simulink model "double_PID_actual"  (R2024b)
settings: Solver=VariableStepAuto  StartTime=0  StopTime=3  FixedStep=0.0000001
undefined symbols (not defined in the file or in its folder): DiscIntNeverNeededParam
libraries: simulink x6
settings Model: Creator=kentl  LastModifiedBy=kentliukx

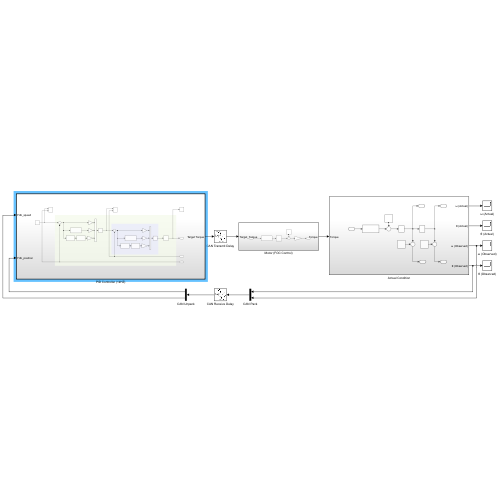
[thumbnail: Simulink's stored preview of the top-level diagram]
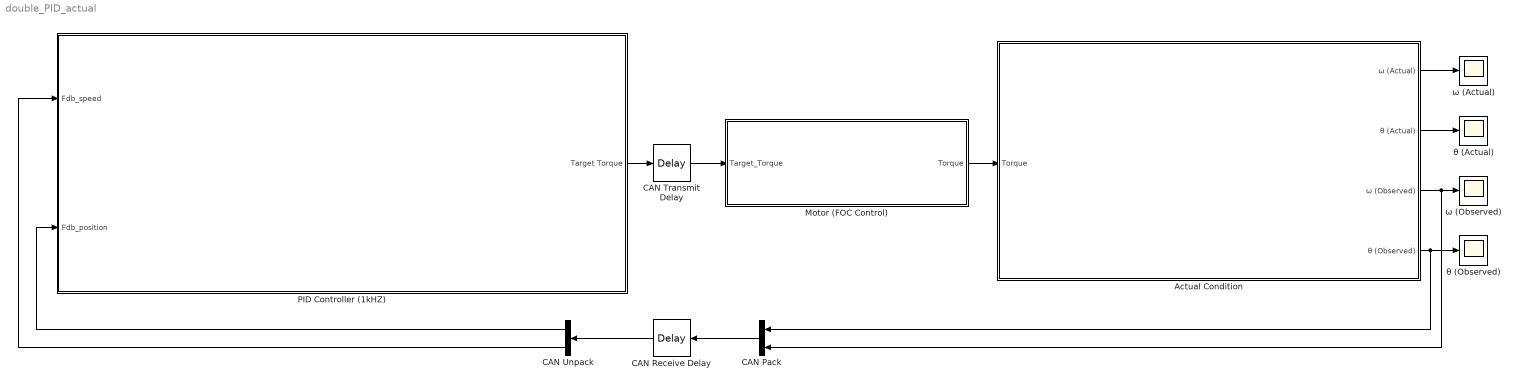
== system double_PID_actual ==
  "Actual Condition " : Subsystem
  CAN Pack : Mux  Inputs=2
  CAN Receive Delay : TransportDelay  DelayTime=0.001
  CAN Transmit Delay : TransportDelay  DelayTime=0.001
  CAN Unpack : Demux  Outputs=2
  "Motor (FOC Control) " : Subsystem
  "PID Controller (1kHZ) " : Subsystem  TreatAsAtomicUnit=on  PartitionName=PID  SystemSampleTime=0.001
  θ (Actual) : Scope
  θ (Observed) : Scope
  ω (Actual) : Scope
  ω (Observed) : Scope
  wires:
  CAN Pack/1 -> CAN Receive Delay/1
  CAN Receive Delay/1 -> CAN Unpack/1
  CAN Unpack/2 -> "PID Controller (1kHZ) "/1(Fdb_speed)
  CAN Unpack/1 -> "PID Controller (1kHZ) "/2(Fdb_position)
  "PID Controller (1kHZ) "/1(Target Torque) -> CAN Transmit Delay/1
  CAN Transmit Delay/1 -> "Motor (FOC Control) "/1(Target_Torque)
  "Actual Condition "/1(ω (Actual)) -> ω (Actual)/1
  "Actual Condition "/2(θ (Actual)) -> θ (Actual)/1
  "Actual Condition "/3(ω (Observed)) -> ω (Observed)/1, CAN Pack/2
  "Actual Condition "/4(θ (Observed)) -> θ (Observed)/1, CAN Pack/1
  "Motor (FOC Control) "/1(Torque) -> "Actual Condition "/1(Torque)

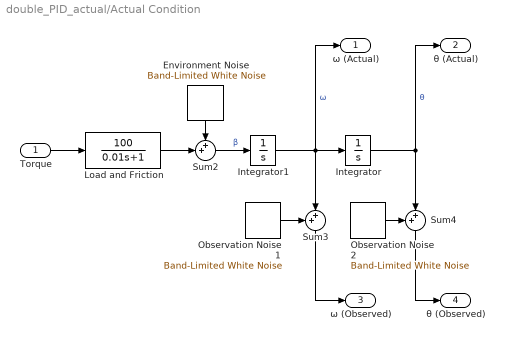
== system double_PID_actual/Actual Condition  ==
  Torque : Inport
  Environment Noise : simulink/Sources/Band-Limited White Noise  Cov=0.1  Ts=0.001  seed=[2331]
  Integrator : Integrator
  Integrator1 : Integrator
  Load and Friction : TransferFcn  Numerator=[100]  Denominator=[0.01 1]
  Observation Noise 1 : simulink/Sources/Band-Limited White Noise  Cov=0.0000001  Ts=0.001  seed=[23341]
  Observation Noise 2 : simulink/Sources/Band-Limited White Noise  Cov=0.0000001  Ts=0.001  seed=[23340]
  Sum2 : Sum  Inputs=++|
  Sum3 : Sum  Inputs=++|
  Sum4 : Sum  Inputs=++|
  ω (Actual) : Outport
  θ (Actual) : Outport  Port=2
  ω (Observed) : Outport  Port=3
  θ (Observed) : Outport  Port=4
  wires:
  Environment Noise/1 -> Sum2/1
  Integrator/1 -> θ (Actual)/1, Sum4/2  "θ"
  Observation Noise 1/1 -> Sum3/1
  Observation Noise 2/1 -> Sum4/1
  Sum3/1 -> ω (Observed)/1
  Sum4/1 -> θ (Observed)/1
  Integrator1/1 -> ω (Actual)/1, Integrator/1, Sum3/2  "ω"
  Sum2/1 -> Integrator1/1  "β"
  Load and Friction/1 -> Sum2/2
  Torque/1 -> Load and Friction/1

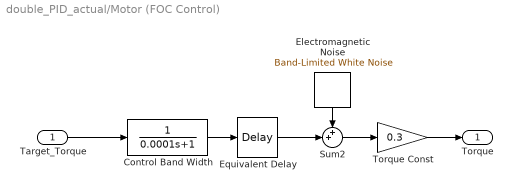
== system double_PID_actual/Motor (FOC Control)  ==
  Target_Torque : Inport
  Control Band Width : TransferFcn  Denominator=[0.0001 1]
  Electromagnetic Noise : simulink/Sources/Band-Limited White Noise  Cov=0.0001  Ts=0.001  seed=[23341]
  Equivalent Delay : TransportDelay  DelayTime=0.001
  Sum2 : Sum  Inputs=++|
  Torque Const : Gain  Gain=0.3
  Torque : Outport
  wires:
  Control Band Width/1 -> Equivalent Delay/1
  Target_Torque/1 -> Control Band Width/1
  Torque Const/1 -> Torque/1
  Equivalent Delay/1 -> Sum2/2
  Sum2/1 -> Torque Const/1
  Electromagnetic Noise/1 -> Sum2/1

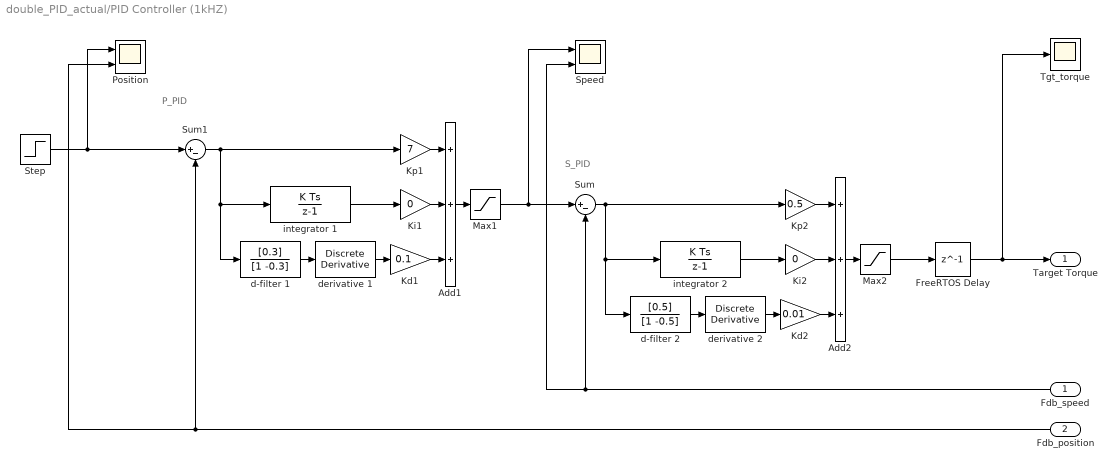
== system double_PID_actual/PID Controller (1kHZ)  ==
  note: P_PID
  note: S_PID
  Fdb_speed : Inport
  Fdb_position : Inport  Port=2
  Add1 : Sum  Inputs=+++
  Add2 : Sum  Inputs=+++
  FreeRTOS Delay : Delay  DelayLength=1
  Kd1 : Gain  Gain=0.1
  Kd2 : Gain  Gain=0.01
  Ki1 : Gain  Gain=0
  Ki2 : Gain  Gain=0
  Kp1 : Gain  Gain=7
  Kp2 : Gain  Gain=0.5
  Max1 : Saturate  UpperLimit=360  LowerLimit=-360
  Max2 : Saturate  UpperLimit=20  LowerLimit=-20
  Position : Scope  NumInputPorts=2
  Speed : Scope  NumInputPorts=2
  Step : Step  After=10
  Sum : Sum  Inputs=|+-
  Sum1 : Sum  Inputs=|+-
  Tgt_torque : Scope
  d-filter 1 : DiscreteFilter  Numerator=[0.3]  Denominator=[1 -0.3]
  d-filter 2 : DiscreteFilter  Numerator=[0.5]  Denominator=[1 -0.5]
  derivative 1 : simulink/Discrete/Discrete Derivative  gainval=1.0  ICPrevScaledInput=0.0  OutMin=[]  OutMax=[]  OutDataType=fixdt(1, 16)  OutScaling=2^-10  DoSatur=off
  derivative 2 : simulink/Discrete/Discrete Derivative  gainval=1.0  ICPrevScaledInput=0.0  OutMin=[]  OutMax=[]  OutDataType=fixdt(1, 16)  OutScaling=2^-10  DoSatur=off
  integrator 1 : DiscreteIntegrator  SampleTime=-1  LimitOutput=on  UpperSaturationLimit=20  LowerSaturationLimit=-20  ICPrevOutput=DiscIntNeverNeededParam  ICPrevScaledInput=DiscIntNeverNeededParam
  integrator 2 : DiscreteIntegrator  SampleTime=-1  LimitOutput=on  UpperSaturationLimit=20  LowerSaturationLimit=-20  ICPrevOutput=DiscIntNeverNeededParam  ICPrevScaledInput=DiscIntNeverNeededParam
  Target Torque : Outport
  wires:
  Step/1 -> Position/1, Sum1/1
  Max2/1 -> FreeRTOS Delay/1
  Kp1/1 -> Add1/1
  Sum1/1 -> d-filter 1/1, integrator 1/1, Kp1/1
  Add1/1 -> Max1/1
  Fdb_speed/1 -> Speed/2, Sum/2
  Fdb_position/1 -> Position/2, Sum1/2
  Ki1/1 -> Add1/2
  derivative 1/1 -> Kd1/1
  integrator 1/1 -> Ki1/1
  Kd1/1 -> Add1/3
  Add2/1 -> Max2/1
  d-filter 1/1 -> derivative 1/1
  Kd2/1 -> Add2/3
  Ki2/1 -> Add2/2
  Sum/1 -> d-filter 2/1, integrator 2/1, Kp2/1
  Kp2/1 -> Add2/1
  d-filter 2/1 -> derivative 2/1
  derivative 2/1 -> Kd2/1
  integrator 2/1 -> Ki2/1
  FreeRTOS Delay/1 -> Tgt_torque/1, Target Torque/1
  Max1/1 -> Speed/1, Sum/1
